simulink model "TB32_A25R_ClampMix"  (R2025a)
settings: Solver=FixedStepDiscrete  StartTime=0  StopTime=TB.t_end  FixedStep=TB.dt  RelTol=1e-3
InitFcn:
  | % 모델과 같은 폴더의 초기화 스크립트를 실행해 P(설계 파라미터)와 TB(시험 조건)를 만든다.
  | run(fullfile(fileparts(get_param(bdroot, 'FileName')), 'TB32_init.m'));
values from neighbouring files (symbols this model uses):
  TB = struct()    [TB32_init.m]    (also in run_TB32.m = evalin('base', 'TB'))
libraries: fl_lib x227, nesl_utility x83
(part 3 of 4)

== system TB32_A25R_ClampMix/StageC_Regulated/Primary_Bridge ==
  note: Stage C 1차 풀브리지(650 V GaN 2병렬): 1차가 보낼 때 250 kHz 50 % 상보 + 데드타임 t_dp, 2차가 보낼 때는 꺼 두고 다이오드 정류(경부하 두 브리지 구동 모드에서는 같은 위상)
  Q1_leg1_high : Subsystem  mask(PRISM-Hub switch cell){Ron=TB.CP.Ron, Goff=TB.CP.Goff, Vf=TB.CP.Vf, Rd=TB.CP.Rd, Goffd=TB.CP.Goffd, Coss=TB.CP.Coss}
      mask prompts: Ron "도통 저항 R_on [Ohm]"; Goff "차단 컨덕턴스 G_off [S]"; Vf "다이오드 순방향 전압 Vf [V]"; Rd "다이오드 도통 저항 R_d [Ohm]"; Goffd "다이오드 차단 컨덕턴스 [S]"; Coss "출력용량 C_oss [F]"
      mask help: 전력 반도체 스위치 셀 Q1_leg1_high. 게이트 태그 gC_Q1.
      settings: AttributesFormatString=gate: gC_Q1
      mask Display:
      | plot([0.50 0.50 ],[0.95 0.65 ],[0.50 0.74 ],[0.65 0.35 ],[0.50 0.50 ],[0.35 0.05 ]);
      | plot([0.50 0.20 0.20 ],[0.80 0.80 0.58 ],[0.20 0.20 0.50 ],[0.42 0.20 0.20 ]);
      | plot([0.20 0.10 0.30 0.20 ],[0.58 0.42 0.42 0.58 ],[0.10 0.30 ],[0.58 0.58 ]);
      | port_label('LConn',1,'D');
      | port_label('RConn',1,'S');
  Q2_leg1_low : Subsystem  mask(PRISM-Hub switch cell){Ron=TB.CP.Ron, Goff=TB.CP.Goff, Vf=TB.CP.Vf, Rd=TB.CP.Rd, Goffd=TB.CP.Goffd, Coss=TB.CP.Coss}
      mask prompts: Ron "도통 저항 R_on [Ohm]"; Goff "차단 컨덕턴스 G_off [S]"; Vf "다이오드 순방향 전압 Vf [V]"; Rd "다이오드 도통 저항 R_d [Ohm]"; Goffd "다이오드 차단 컨덕턴스 [S]"; Coss "출력용량 C_oss [F]"
      mask help: 전력 반도체 스위치 셀 Q2_leg1_low. 게이트 태그 gC_Q2.
      settings: AttributesFormatString=gate: gC_Q2
      mask Display:
      | plot([0.50 0.50 ],[0.95 0.65 ],[0.50 0.74 ],[0.65 0.35 ],[0.50 0.50 ],[0.35 0.05 ]);
      | plot([0.50 0.20 0.20 ],[0.80 0.80 0.58 ],[0.20 0.20 0.50 ],[0.42 0.20 0.20 ]);
      | plot([0.20 0.10 0.30 0.20 ],[0.58 0.42 0.42 0.58 ],[0.10 0.30 ],[0.58 0.58 ]);
      | port_label('LConn',1,'D');
      | port_label('RConn',1,'S');
  Q3_leg2_high : Subsystem  mask(PRISM-Hub switch cell){Ron=TB.CP.Ron, Goff=TB.CP.Goff, Vf=TB.CP.Vf, Rd=TB.CP.Rd, Goffd=TB.CP.Goffd, Coss=TB.CP.Coss}
      mask prompts: Ron "도통 저항 R_on [Ohm]"; Goff "차단 컨덕턴스 G_off [S]"; Vf "다이오드 순방향 전압 Vf [V]"; Rd "다이오드 도통 저항 R_d [Ohm]"; Goffd "다이오드 차단 컨덕턴스 [S]"; Coss "출력용량 C_oss [F]"
      mask help: 전력 반도체 스위치 셀 Q3_leg2_high. 게이트 태그 gC_Q3.
      settings: AttributesFormatString=gate: gC_Q3
      mask Display:
      | plot([0.50 0.50 ],[0.95 0.65 ],[0.50 0.74 ],[0.65 0.35 ],[0.50 0.50 ],[0.35 0.05 ]);
      | plot([0.50 0.20 0.20 ],[0.80 0.80 0.58 ],[0.20 0.20 0.50 ],[0.42 0.20 0.20 ]);
      | plot([0.20 0.10 0.30 0.20 ],[0.58 0.42 0.42 0.58 ],[0.10 0.30 ],[0.58 0.58 ]);
      | port_label('LConn',1,'D');
      | port_label('RConn',1,'S');
  Q4_leg2_low : Subsystem  mask(PRISM-Hub switch cell){Ron=TB.CP.Ron, Goff=TB.CP.Goff, Vf=TB.CP.Vf, Rd=TB.CP.Rd, Goffd=TB.CP.Goffd, Coss=TB.CP.Coss}
      mask prompts: Ron "도통 저항 R_on [Ohm]"; Goff "차단 컨덕턴스 G_off [S]"; Vf "다이오드 순방향 전압 Vf [V]"; Rd "다이오드 도통 저항 R_d [Ohm]"; Goffd "다이오드 차단 컨덕턴스 [S]"; Coss "출력용량 C_oss [F]"
      mask help: 전력 반도체 스위치 셀 Q4_leg2_low. 게이트 태그 gC_Q4.
      settings: AttributesFormatString=gate: gC_Q4
      mask Display:
      | plot([0.50 0.50 ],[0.95 0.65 ],[0.50 0.74 ],[0.65 0.35 ],[0.50 0.50 ],[0.35 0.05 ]);
      | plot([0.50 0.20 0.20 ],[0.80 0.80 0.58 ],[0.20 0.20 0.50 ],[0.42 0.20 0.20 ]);
      | plot([0.20 0.10 0.30 0.20 ],[0.58 0.42 0.42 0.58 ],[0.10 0.30 ],[0.58 0.58 ]);
      | port_label('LConn',1,'D');
      | port_label('RConn',1,'S');
  DC_P : PMIOPort  Side=Left
  DC_N : PMIOPort  Port=2  Side=Left
  AC1 : PMIOPort  Port=3  Side=Right
  AC2 : PMIOPort  Port=4  Side=Right
  connections:
  Q1_leg1_high/LConn1 -- DC_P/RConn1 -- Q3_leg2_high/LConn1
  Q2_leg1_low/LConn1 -- Q1_leg1_high/RConn1 -- AC1/RConn1
  Q4_leg2_low/LConn1 -- Q3_leg2_high/RConn1 -- AC2/RConn1
  DC_N/RConn1 -- Q2_leg1_low/RConn1 -- Q4_leg2_low/RConn1

== system TB32_A25R_ClampMix/StageC_Regulated/SB_H_high ==
  note: 스위치 셀: 이상 스위치(R_on, G_off) + 역병렬 바디 다이오드(Vf, R_d) + 출력용량 C_oss
      | 게이트: 전역 태그 "gS_BH" (> 0.5 이면 도통)
  C_oss : fl_lib/Electrical/Electrical Elements/Capacitor  c=Coss F  r=1e-6 Ohm  g=0 1/Ohm  i_specify=off  i_priority=None  i=0 A  i_nominal_specify=off  i_nominal_value=1  i_nominal_unit=A  v_specify=off  v_priority=None  v=0 V  v_nominal_specify=off  v_nominal_value=1  v_nominal_unit=V  vc_specify=off  vc_priority=High  vc=0 V  vc_nominal_specify=off  vc_nominal_value=1  vc_nominal_unit=V
  D_body : fl_lib/Electrical/Electrical Elements/Diode  Vf=Vf V  Ron=Rd Ohm  Goff=Goffd 1/Ohm  i_specify=off  i_priority=None  i=0 A  i_nominal_specify=off  i_nominal_value=1  i_nominal_unit=A  v_specify=off  v_priority=None  v=0 V  v_nominal_specify=off  v_nominal_value=1  v_nominal_unit=V
  Gate_PS : nesl_utility/Simulink-PS Converter  PhysicalDomain=network_engine_domain  SubClassName=ps_input  LeftPortType=input  RightPortType=output  PseudoPeriodic=off  Frequencies=[]  NoiseDistribution=none  NoiseParameters=[]  Unit=1  AffineConversion=off  FilteringAndDerivatives=zero  SimscapeFilterOrder=1  InputFilterTimeConstant=0.001  UdotUserProvided=0
  SW : fl_lib/Electrical/Electrical Elements/Switch  R_closed=Ron Ohm  G_open=Goff 1/Ohm  Threshold=0.5  i_specify=off  i_priority=None  i=0 A  i_nominal_specify=off  i_nominal_value=1  i_nominal_unit=A  v_specify=off  v_priority=None  v=0 V  v_nominal_specify=off  v_nominal_value=1  v_nominal_unit=V
  D : PMIOPort  Side=Left
  S : PMIOPort  Port=2  Side=Right
  wires:
  [gS_BH] -> Gate_PS/1
  connections:
  Gate_PS/RConn1 -- SW/RConn1
  SW/LConn1 -- D/RConn1 -- D_body/RConn1 -- C_oss/LConn1
  SW/RConn2 -- D_body/LConn1 -- S/RConn1 -- C_oss/RConn1

== system TB32_A25R_ClampMix/StageC_Regulated/SB_L_low ==
  note: 스위치 셀: 이상 스위치(R_on, G_off) + 역병렬 바디 다이오드(Vf, R_d) + 출력용량 C_oss
      | 게이트: 전역 태그 "gS_BL" (> 0.5 이면 도통)
  C_oss : fl_lib/Electrical/Electrical Elements/Capacitor  c=Coss F  r=1e-6 Ohm  g=0 1/Ohm  i_specify=off  i_priority=None  i=0 A  i_nominal_specify=off  i_nominal_value=1  i_nominal_unit=A  v_specify=off  v_priority=None  v=0 V  v_nominal_specify=off  v_nominal_value=1  v_nominal_unit=V  vc_specify=off  vc_priority=High  vc=0 V  vc_nominal_specify=off  vc_nominal_value=1  vc_nominal_unit=V
  D_body : fl_lib/Electrical/Electrical Elements/Diode  Vf=Vf V  Ron=Rd Ohm  Goff=Goffd 1/Ohm  i_specify=off  i_priority=None  i=0 A  i_nominal_specify=off  i_nominal_value=1  i_nominal_unit=A  v_specify=off  v_priority=None  v=0 V  v_nominal_specify=off  v_nominal_value=1  v_nominal_unit=V
  Gate_PS : nesl_utility/Simulink-PS Converter  PhysicalDomain=network_engine_domain  SubClassName=ps_input  LeftPortType=input  RightPortType=output  PseudoPeriodic=off  Frequencies=[]  NoiseDistribution=none  NoiseParameters=[]  Unit=1  AffineConversion=off  FilteringAndDerivatives=zero  SimscapeFilterOrder=1  InputFilterTimeConstant=0.001  UdotUserProvided=0
  SW : fl_lib/Electrical/Electrical Elements/Switch  R_closed=Ron Ohm  G_open=Goff 1/Ohm  Threshold=0.5  i_specify=off  i_priority=None  i=0 A  i_nominal_specify=off  i_nominal_value=1  i_nominal_unit=A  v_specify=off  v_priority=None  v=0 V  v_nominal_specify=off  v_nominal_value=1  v_nominal_unit=V
  D : PMIOPort  Side=Left
  S : PMIOPort  Port=2  Side=Right
  wires:
  [gS_BL] -> Gate_PS/1
  connections:
  Gate_PS/RConn1 -- SW/RConn1
  SW/LConn1 -- D/RConn1 -- D_body/RConn1 -- C_oss/LConn1
  SW/RConn2 -- D_body/LConn1 -- S/RConn1 -- C_oss/RConn1

== system TB32_A25R_ClampMix/StageC_Regulated/Secondary_Bridge ==
  note: Stage C 2차 풀브리지(150 V GaN 2병렬): 1차가 보낼 때는 꺼 두고 다이오드 정류(이상 동기정류 근사), 2차가 보낼 때 250 kHz + 데드타임 t_ds
  S1_leg1_high : Subsystem  mask(PRISM-Hub switch cell){Ron=TB.CS.Ron, Goff=TB.CS.Goff, Vf=TB.CS.Vf, Rd=TB.CS.Rd, Goffd=TB.CS.Goffd, Coss=TB.CS.Coss}
      mask prompts: Ron "도통 저항 R_on [Ohm]"; Goff "차단 컨덕턴스 G_off [S]"; Vf "다이오드 순방향 전압 Vf [V]"; Rd "다이오드 도통 저항 R_d [Ohm]"; Goffd "다이오드 차단 컨덕턴스 [S]"; Coss "출력용량 C_oss [F]"
      mask help: 전력 반도체 스위치 셀 S1_leg1_high. 게이트 태그 gC_S1.
      settings: AttributesFormatString=gate: gC_S1
      mask Display:
      | plot([0.50 0.50 ],[0.95 0.65 ],[0.50 0.74 ],[0.65 0.35 ],[0.50 0.50 ],[0.35 0.05 ]);
      | plot([0.50 0.20 0.20 ],[0.80 0.80 0.58 ],[0.20 0.20 0.50 ],[0.42 0.20 0.20 ]);
      | plot([0.20 0.10 0.30 0.20 ],[0.58 0.42 0.42 0.58 ],[0.10 0.30 ],[0.58 0.58 ]);
      | port_label('LConn',1,'D');
      | port_label('RConn',1,'S');
  S2_leg1_low : Subsystem  mask(PRISM-Hub switch cell){Ron=TB.CS.Ron, Goff=TB.CS.Goff, Vf=TB.CS.Vf, Rd=TB.CS.Rd, Goffd=TB.CS.Goffd, Coss=TB.CS.Coss}
      mask prompts: Ron "도통 저항 R_on [Ohm]"; Goff "차단 컨덕턴스 G_off [S]"; Vf "다이오드 순방향 전압 Vf [V]"; Rd "다이오드 도통 저항 R_d [Ohm]"; Goffd "다이오드 차단 컨덕턴스 [S]"; Coss "출력용량 C_oss [F]"
      mask help: 전력 반도체 스위치 셀 S2_leg1_low. 게이트 태그 gC_S2.
      settings: AttributesFormatString=gate: gC_S2
      mask Display:
      | plot([0.50 0.50 ],[0.95 0.65 ],[0.50 0.74 ],[0.65 0.35 ],[0.50 0.50 ],[0.35 0.05 ]);
      | plot([0.50 0.20 0.20 ],[0.80 0.80 0.58 ],[0.20 0.20 0.50 ],[0.42 0.20 0.20 ]);
      | plot([0.20 0.10 0.30 0.20 ],[0.58 0.42 0.42 0.58 ],[0.10 0.30 ],[0.58 0.58 ]);
      | port_label('LConn',1,'D');
      | port_label('RConn',1,'S');
  S3_leg2_high : Subsystem  mask(PRISM-Hub switch cell){Ron=TB.CS.Ron, Goff=TB.CS.Goff, Vf=TB.CS.Vf, Rd=TB.CS.Rd, Goffd=TB.CS.Goffd, Coss=TB.CS.Coss}
      mask prompts: Ron "도통 저항 R_on [Ohm]"; Goff "차단 컨덕턴스 G_off [S]"; Vf "다이오드 순방향 전압 Vf [V]"; Rd "다이오드 도통 저항 R_d [Ohm]"; Goffd "다이오드 차단 컨덕턴스 [S]"; Coss "출력용량 C_oss [F]"
      mask help: 전력 반도체 스위치 셀 S3_leg2_high. 게이트 태그 gC_S3.
      settings: AttributesFormatString=gate: gC_S3
      mask Display:
      | plot([0.50 0.50 ],[0.95 0.65 ],[0.50 0.74 ],[0.65 0.35 ],[0.50 0.50 ],[0.35 0.05 ]);
      | plot([0.50 0.20 0.20 ],[0.80 0.80 0.58 ],[0.20 0.20 0.50 ],[0.42 0.20 0.20 ]);
      | plot([0.20 0.10 0.30 0.20 ],[0.58 0.42 0.42 0.58 ],[0.10 0.30 ],[0.58 0.58 ]);
      | port_label('LConn',1,'D');
      | port_label('RConn',1,'S');
  S4_leg2_low : Subsystem  mask(PRISM-Hub switch cell){Ron=TB.CS.Ron, Goff=TB.CS.Goff, Vf=TB.CS.Vf, Rd=TB.CS.Rd, Goffd=TB.CS.Goffd, Coss=TB.CS.Coss}
      mask prompts: Ron "도통 저항 R_on [Ohm]"; Goff "차단 컨덕턴스 G_off [S]"; Vf "다이오드 순방향 전압 Vf [V]"; Rd "다이오드 도통 저항 R_d [Ohm]"; Goffd "다이오드 차단 컨덕턴스 [S]"; Coss "출력용량 C_oss [F]"
      mask help: 전력 반도체 스위치 셀 S4_leg2_low. 게이트 태그 gC_S4.
      settings: AttributesFormatString=gate: gC_S4
      mask Display:
      | plot([0.50 0.50 ],[0.95 0.65 ],[0.50 0.74 ],[0.65 0.35 ],[0.50 0.50 ],[0.35 0.05 ]);
      | plot([0.50 0.20 0.20 ],[0.80 0.80 0.58 ],[0.20 0.20 0.50 ],[0.42 0.20 0.20 ]);
      | plot([0.20 0.10 0.30 0.20 ],[0.58 0.42 0.42 0.58 ],[0.10 0.30 ],[0.58 0.58 ]);
      | port_label('LConn',1,'D');
      | port_label('RConn',1,'S');
  DC_P : PMIOPort  Side=Left
  DC_N : PMIOPort  Port=2  Side=Left
  AC1 : PMIOPort  Port=3  Side=Right
  AC2 : PMIOPort  Port=4  Side=Right
  connections:
  S1_leg1_high/LConn1 -- DC_P/RConn1 -- S3_leg2_high/LConn1
  S2_leg1_low/LConn1 -- S1_leg1_high/RConn1 -- AC1/RConn1
  S4_leg2_low/LConn1 -- S3_leg2_high/RConn1 -- AC2/RConn1
  DC_N/RConn1 -- S2_leg1_low/RConn1 -- S4_leg2_low/RConn1

== system TB32_A25R_ClampMix/StageA_Module1/StageA_Phase1/S1_VIN_A ==
  note: 스위치 셀: 이상 스위치(R_on, G_off) + 역병렬 바디 다이오드(Vf, R_d) + 출력용량 C_oss
      | 게이트: 전역 태그 "gA_P1_S1" (> 0.5 이면 도통)
  C_oss : fl_lib/Electrical/Electrical Elements/Capacitor  c=Coss F  r=1e-6 Ohm  g=0 1/Ohm  i_specify=off  i_priority=None  i=0 A  i_nominal_specify=off  i_nominal_value=1  i_nominal_unit=A  v_specify=off  v_priority=None  v=0 V  v_nominal_specify=off  v_nominal_value=1  v_nominal_unit=V  vc_specify=off  vc_priority=High  vc=0 V  vc_nominal_specify=off  vc_nominal_value=1  vc_nominal_unit=V
  D_body : fl_lib/Electrical/Electrical Elements/Diode  Vf=Vf V  Ron=Rd Ohm  Goff=Goffd 1/Ohm  i_specify=off  i_priority=None  i=0 A  i_nominal_specify=off  i_nominal_value=1  i_nominal_unit=A  v_specify=off  v_priority=None  v=0 V  v_nominal_specify=off  v_nominal_value=1  v_nominal_unit=V
  Gate_PS : nesl_utility/Simulink-PS Converter  PhysicalDomain=network_engine_domain  SubClassName=ps_input  LeftPortType=input  RightPortType=output  PseudoPeriodic=off  Frequencies=[]  NoiseDistribution=none  NoiseParameters=[]  Unit=1  AffineConversion=off  FilteringAndDerivatives=zero  SimscapeFilterOrder=1  InputFilterTimeConstant=0.001  UdotUserProvided=0
  SW : fl_lib/Electrical/Electrical Elements/Switch  R_closed=Ron Ohm  G_open=Goff 1/Ohm  Threshold=0.5  i_specify=off  i_priority=None  i=0 A  i_nominal_specify=off  i_nominal_value=1  i_nominal_unit=A  v_specify=off  v_priority=None  v=0 V  v_nominal_specify=off  v_nominal_value=1  v_nominal_unit=V
  D : PMIOPort  Side=Left
  S : PMIOPort  Port=2  Side=Right
  wires:
  [gA_P1_S1] -> Gate_PS/1
  connections:
  Gate_PS/RConn1 -- SW/RConn1
  SW/LConn1 -- D/RConn1 -- D_body/RConn1 -- C_oss/LConn1
  SW/RConn2 -- D_body/LConn1 -- S/RConn1 -- C_oss/RConn1

== system TB32_A25R_ClampMix/StageA_Module1/StageA_Phase1/S2_A_VOUT ==
  note: 스위치 셀: 이상 스위치(R_on, G_off) + 역병렬 바디 다이오드(Vf, R_d) + 출력용량 C_oss
      | 게이트: 전역 태그 "gA_P1_S2" (> 0.5 이면 도통)
  C_oss : fl_lib/Electrical/Electrical Elements/Capacitor  c=Coss F  r=1e-6 Ohm  g=0 1/Ohm  i_specify=off  i_priority=None  i=0 A  i_nominal_specify=off  i_nominal_value=1  i_nominal_unit=A  v_specify=off  v_priority=None  v=0 V  v_nominal_specify=off  v_nominal_value=1  v_nominal_unit=V  vc_specify=off  vc_priority=High  vc=0 V  vc_nominal_specify=off  vc_nominal_value=1  vc_nominal_unit=V
  D_body : fl_lib/Electrical/Electrical Elements/Diode  Vf=Vf V  Ron=Rd Ohm  Goff=Goffd 1/Ohm  i_specify=off  i_priority=None  i=0 A  i_nominal_specify=off  i_nominal_value=1  i_nominal_unit=A  v_specify=off  v_priority=None  v=0 V  v_nominal_specify=off  v_nominal_value=1  v_nominal_unit=V
  Gate_PS : nesl_utility/Simulink-PS Converter  PhysicalDomain=network_engine_domain  SubClassName=ps_input  LeftPortType=input  RightPortType=output  PseudoPeriodic=off  Frequencies=[]  NoiseDistribution=none  NoiseParameters=[]  Unit=1  AffineConversion=off  FilteringAndDerivatives=zero  SimscapeFilterOrder=1  InputFilterTimeConstant=0.001  UdotUserProvided=0
  SW : fl_lib/Electrical/Electrical Elements/Switch  R_closed=Ron Ohm  G_open=Goff 1/Ohm  Threshold=0.5  i_specify=off  i_priority=None  i=0 A  i_nominal_specify=off  i_nominal_value=1  i_nominal_unit=A  v_specify=off  v_priority=None  v=0 V  v_nominal_specify=off  v_nominal_value=1  v_nominal_unit=V
  D : PMIOPort  Side=Left
  S : PMIOPort  Port=2  Side=Right
  wires:
  [gA_P1_S2] -> Gate_PS/1
  connections:
  Gate_PS/RConn1 -- SW/RConn1
  SW/LConn1 -- D/RConn1 -- D_body/RConn1 -- C_oss/LConn1
  SW/RConn2 -- D_body/LConn1 -- S/RConn1 -- C_oss/RConn1

== system TB32_A25R_ClampMix/StageA_Module1/StageA_Phase1/S3_VOUT_B ==
  note: 스위치 셀: 이상 스위치(R_on, G_off) + 역병렬 바디 다이오드(Vf, R_d) + 출력용량 C_oss
      | 게이트: 전역 태그 "gA_P1_S3" (> 0.5 이면 도통)
  C_oss : fl_lib/Electrical/Electrical Elements/Capacitor  c=Coss F  r=1e-6 Ohm  g=0 1/Ohm  i_specify=off  i_priority=None  i=0 A  i_nominal_specify=off  i_nominal_value=1  i_nominal_unit=A  v_specify=off  v_priority=None  v=0 V  v_nominal_specify=off  v_nominal_value=1  v_nominal_unit=V  vc_specify=off  vc_priority=High  vc=0 V  vc_nominal_specify=off  vc_nominal_value=1  vc_nominal_unit=V
  D_body : fl_lib/Electrical/Electrical Elements/Diode  Vf=Vf V  Ron=Rd Ohm  Goff=Goffd 1/Ohm  i_specify=off  i_priority=None  i=0 A  i_nominal_specify=off  i_nominal_value=1  i_nominal_unit=A  v_specify=off  v_priority=None  v=0 V  v_nominal_specify=off  v_nominal_value=1  v_nominal_unit=V
  Gate_PS : nesl_utility/Simulink-PS Converter  PhysicalDomain=network_engine_domain  SubClassName=ps_input  LeftPortType=input  RightPortType=output  PseudoPeriodic=off  Frequencies=[]  NoiseDistribution=none  NoiseParameters=[]  Unit=1  AffineConversion=off  FilteringAndDerivatives=zero  SimscapeFilterOrder=1  InputFilterTimeConstant=0.001  UdotUserProvided=0
  SW : fl_lib/Electrical/Electrical Elements/Switch  R_closed=Ron Ohm  G_open=Goff 1/Ohm  Threshold=0.5  i_specify=off  i_priority=None  i=0 A  i_nominal_specify=off  i_nominal_value=1  i_nominal_unit=A  v_specify=off  v_priority=None  v=0 V  v_nominal_specify=off  v_nominal_value=1  v_nominal_unit=V
  D : PMIOPort  Side=Left
  S : PMIOPort  Port=2  Side=Right
  wires:
  [gA_P1_S3] -> Gate_PS/1
  connections:
  Gate_PS/RConn1 -- SW/RConn1
  SW/LConn1 -- D/RConn1 -- D_body/RConn1 -- C_oss/LConn1
  SW/RConn2 -- D_body/LConn1 -- S/RConn1 -- C_oss/RConn1

== system TB32_A25R_ClampMix/StageA_Module1/StageA_Phase1/S4_B_GND ==
  note: 스위치 셀: 이상 스위치(R_on, G_off) + 역병렬 바디 다이오드(Vf, R_d) + 출력용량 C_oss
      | 게이트: 전역 태그 "gA_P1_S4" (> 0.5 이면 도통)
  C_oss : fl_lib/Electrical/Electrical Elements/Capacitor  c=Coss F  r=1e-6 Ohm  g=0 1/Ohm  i_specify=off  i_priority=None  i=0 A  i_nominal_specify=off  i_nominal_value=1  i_nominal_unit=A  v_specify=off  v_priority=None  v=0 V  v_nominal_specify=off  v_nominal_value=1  v_nominal_unit=V  vc_specify=off  vc_priority=High  vc=0 V  vc_nominal_specify=off  vc_nominal_value=1  vc_nominal_unit=V
  D_body : fl_lib/Electrical/Electrical Elements/Diode  Vf=Vf V  Ron=Rd Ohm  Goff=Goffd 1/Ohm  i_specify=off  i_priority=None  i=0 A  i_nominal_specify=off  i_nominal_value=1  i_nominal_unit=A  v_specify=off  v_priority=None  v=0 V  v_nominal_specify=off  v_nominal_value=1  v_nominal_unit=V
  Gate_PS : nesl_utility/Simulink-PS Converter  PhysicalDomain=network_engine_domain  SubClassName=ps_input  LeftPortType=input  RightPortType=output  PseudoPeriodic=off  Frequencies=[]  NoiseDistribution=none  NoiseParameters=[]  Unit=1  AffineConversion=off  FilteringAndDerivatives=zero  SimscapeFilterOrder=1  InputFilterTimeConstant=0.001  UdotUserProvided=0
  SW : fl_lib/Electrical/Electrical Elements/Switch  R_closed=Ron Ohm  G_open=Goff 1/Ohm  Threshold=0.5  i_specify=off  i_priority=None  i=0 A  i_nominal_specify=off  i_nominal_value=1  i_nominal_unit=A  v_specify=off  v_priority=None  v=0 V  v_nominal_specify=off  v_nominal_value=1  v_nominal_unit=V
  D : PMIOPort  Side=Left
  S : PMIOPort  Port=2  Side=Right
  wires:
  [gA_P1_S4] -> Gate_PS/1
  connections:
  Gate_PS/RConn1 -- SW/RConn1
  SW/LConn1 -- D/RConn1 -- D_body/RConn1 -- C_oss/LConn1
  SW/RConn2 -- D_body/LConn1 -- S/RConn1 -- C_oss/RConn1

== system TB32_A25R_ClampMix/StageA_Module1/StageA_Phase2/S1_VIN_A ==
  note: 스위치 셀: 이상 스위치(R_on, G_off) + 역병렬 바디 다이오드(Vf, R_d) + 출력용량 C_oss
      | 게이트: 전역 태그 "gA_P2_S1" (> 0.5 이면 도통)
  C_oss : fl_lib/Electrical/Electrical Elements/Capacitor  c=Coss F  r=1e-6 Ohm  g=0 1/Ohm  i_specify=off  i_priority=None  i=0 A  i_nominal_specify=off  i_nominal_value=1  i_nominal_unit=A  v_specify=off  v_priority=None  v=0 V  v_nominal_specify=off  v_nominal_value=1  v_nominal_unit=V  vc_specify=off  vc_priority=High  vc=0 V  vc_nominal_specify=off  vc_nominal_value=1  vc_nominal_unit=V
  D_body : fl_lib/Electrical/Electrical Elements/Diode  Vf=Vf V  Ron=Rd Ohm  Goff=Goffd 1/Ohm  i_specify=off  i_priority=None  i=0 A  i_nominal_specify=off  i_nominal_value=1  i_nominal_unit=A  v_specify=off  v_priority=None  v=0 V  v_nominal_specify=off  v_nominal_value=1  v_nominal_unit=V
  Gate_PS : nesl_utility/Simulink-PS Converter  PhysicalDomain=network_engine_domain  SubClassName=ps_input  LeftPortType=input  RightPortType=output  PseudoPeriodic=off  Frequencies=[]  NoiseDistribution=none  NoiseParameters=[]  Unit=1  AffineConversion=off  FilteringAndDerivatives=zero  SimscapeFilterOrder=1  InputFilterTimeConstant=0.001  UdotUserProvided=0
  SW : fl_lib/Electrical/Electrical Elements/Switch  R_closed=Ron Ohm  G_open=Goff 1/Ohm  Threshold=0.5  i_specify=off  i_priority=None  i=0 A  i_nominal_specify=off  i_nominal_value=1  i_nominal_unit=A  v_specify=off  v_priority=None  v=0 V  v_nominal_specify=off  v_nominal_value=1  v_nominal_unit=V
  D : PMIOPort  Side=Left
  S : PMIOPort  Port=2  Side=Right
  wires:
  [gA_P2_S1] -> Gate_PS/1
  connections:
  Gate_PS/RConn1 -- SW/RConn1
  SW/LConn1 -- D/RConn1 -- D_body/RConn1 -- C_oss/LConn1
  SW/RConn2 -- D_body/LConn1 -- S/RConn1 -- C_oss/RConn1

== system TB32_A25R_ClampMix/StageA_Module1/StageA_Phase2/S2_A_VOUT ==
  note: 스위치 셀: 이상 스위치(R_on, G_off) + 역병렬 바디 다이오드(Vf, R_d) + 출력용량 C_oss
      | 게이트: 전역 태그 "gA_P2_S2" (> 0.5 이면 도통)
  C_oss : fl_lib/Electrical/Electrical Elements/Capacitor  c=Coss F  r=1e-6 Ohm  g=0 1/Ohm  i_specify=off  i_priority=None  i=0 A  i_nominal_specify=off  i_nominal_value=1  i_nominal_unit=A  v_specify=off  v_priority=None  v=0 V  v_nominal_specify=off  v_nominal_value=1  v_nominal_unit=V  vc_specify=off  vc_priority=High  vc=0 V  vc_nominal_specify=off  vc_nominal_value=1  vc_nominal_unit=V
  D_body : fl_lib/Electrical/Electrical Elements/Diode  Vf=Vf V  Ron=Rd Ohm  Goff=Goffd 1/Ohm  i_specify=off  i_priority=None  i=0 A  i_nominal_specify=off  i_nominal_value=1  i_nominal_unit=A  v_specify=off  v_priority=None  v=0 V  v_nominal_specify=off  v_nominal_value=1  v_nominal_unit=V
  Gate_PS : nesl_utility/Simulink-PS Converter  PhysicalDomain=network_engine_domain  SubClassName=ps_input  LeftPortType=input  RightPortType=output  PseudoPeriodic=off  Frequencies=[]  NoiseDistribution=none  NoiseParameters=[]  Unit=1  AffineConversion=off  FilteringAndDerivatives=zero  SimscapeFilterOrder=1  InputFilterTimeConstant=0.001  UdotUserProvided=0
  SW : fl_lib/Electrical/Electrical Elements/Switch  R_closed=Ron Ohm  G_open=Goff 1/Ohm  Threshold=0.5  i_specify=off  i_priority=None  i=0 A  i_nominal_specify=off  i_nominal_value=1  i_nominal_unit=A  v_specify=off  v_priority=None  v=0 V  v_nominal_specify=off  v_nominal_value=1  v_nominal_unit=V
  D : PMIOPort  Side=Left
  S : PMIOPort  Port=2  Side=Right
  wires:
  [gA_P2_S2] -> Gate_PS/1
  connections:
  Gate_PS/RConn1 -- SW/RConn1
  SW/LConn1 -- D/RConn1 -- D_body/RConn1 -- C_oss/LConn1
  SW/RConn2 -- D_body/LConn1 -- S/RConn1 -- C_oss/RConn1

== system TB32_A25R_ClampMix/StageA_Module1/StageA_Phase2/S3_VOUT_B ==
  note: 스위치 셀: 이상 스위치(R_on, G_off) + 역병렬 바디 다이오드(Vf, R_d) + 출력용량 C_oss
      | 게이트: 전역 태그 "gA_P2_S3" (> 0.5 이면 도통)
  C_oss : fl_lib/Electrical/Electrical Elements/Capacitor  c=Coss F  r=1e-6 Ohm  g=0 1/Ohm  i_specify=off  i_priority=None  i=0 A  i_nominal_specify=off  i_nominal_value=1  i_nominal_unit=A  v_specify=off  v_priority=None  v=0 V  v_nominal_specify=off  v_nominal_value=1  v_nominal_unit=V  vc_specify=off  vc_priority=High  vc=0 V  vc_nominal_specify=off  vc_nominal_value=1  vc_nominal_unit=V
  D_body : fl_lib/Electrical/Electrical Elements/Diode  Vf=Vf V  Ron=Rd Ohm  Goff=Goffd 1/Ohm  i_specify=off  i_priority=None  i=0 A  i_nominal_specify=off  i_nominal_value=1  i_nominal_unit=A  v_specify=off  v_priority=None  v=0 V  v_nominal_specify=off  v_nominal_value=1  v_nominal_unit=V
  Gate_PS : nesl_utility/Simulink-PS Converter  PhysicalDomain=network_engine_domain  SubClassName=ps_input  LeftPortType=input  RightPortType=output  PseudoPeriodic=off  Frequencies=[]  NoiseDistribution=none  NoiseParameters=[]  Unit=1  AffineConversion=off  FilteringAndDerivatives=zero  SimscapeFilterOrder=1  InputFilterTimeConstant=0.001  UdotUserProvided=0
  SW : fl_lib/Electrical/Electrical Elements/Switch  R_closed=Ron Ohm  G_open=Goff 1/Ohm  Threshold=0.5  i_specify=off  i_priority=None  i=0 A  i_nominal_specify=off  i_nominal_value=1  i_nominal_unit=A  v_specify=off  v_priority=None  v=0 V  v_nominal_specify=off  v_nominal_value=1  v_nominal_unit=V
  D : PMIOPort  Side=Left
  S : PMIOPort  Port=2  Side=Right
  wires:
  [gA_P2_S3] -> Gate_PS/1
  connections:
  Gate_PS/RConn1 -- SW/RConn1
  SW/LConn1 -- D/RConn1 -- D_body/RConn1 -- C_oss/LConn1
  SW/RConn2 -- D_body/LConn1 -- S/RConn1 -- C_oss/RConn1

== system TB32_A25R_ClampMix/StageA_Module1/StageA_Phase2/S4_B_GND ==
  note: 스위치 셀: 이상 스위치(R_on, G_off) + 역병렬 바디 다이오드(Vf, R_d) + 출력용량 C_oss
      | 게이트: 전역 태그 "gA_P2_S4" (> 0.5 이면 도통)
  C_oss : fl_lib/Electrical/Electrical Elements/Capacitor  c=Coss F  r=1e-6 Ohm  g=0 1/Ohm  i_specify=off  i_priority=None  i=0 A  i_nominal_specify=off  i_nominal_value=1  i_nominal_unit=A  v_specify=off  v_priority=None  v=0 V  v_nominal_specify=off  v_nominal_value=1  v_nominal_unit=V  vc_specify=off  vc_priority=High  vc=0 V  vc_nominal_specify=off  vc_nominal_value=1  vc_nominal_unit=V
  D_body : fl_lib/Electrical/Electrical Elements/Diode  Vf=Vf V  Ron=Rd Ohm  Goff=Goffd 1/Ohm  i_specify=off  i_priority=None  i=0 A  i_nominal_specify=off  i_nominal_value=1  i_nominal_unit=A  v_specify=off  v_priority=None  v=0 V  v_nominal_specify=off  v_nominal_value=1  v_nominal_unit=V
  Gate_PS : nesl_utility/Simulink-PS Converter  PhysicalDomain=network_engine_domain  SubClassName=ps_input  LeftPortType=input  RightPortType=output  PseudoPeriodic=off  Frequencies=[]  NoiseDistribution=none  NoiseParameters=[]  Unit=1  AffineConversion=off  FilteringAndDerivatives=zero  SimscapeFilterOrder=1  InputFilterTimeConstant=0.001  UdotUserProvided=0
  SW : fl_lib/Electrical/Electrical Elements/Switch  R_closed=Ron Ohm  G_open=Goff 1/Ohm  Threshold=0.5  i_specify=off  i_priority=None  i=0 A  i_nominal_specify=off  i_nominal_value=1  i_nominal_unit=A  v_specify=off  v_priority=None  v=0 V  v_nominal_specify=off  v_nominal_value=1  v_nominal_unit=V
  D : PMIOPort  Side=Left
  S : PMIOPort  Port=2  Side=Right
  wires:
  [gA_P2_S4] -> Gate_PS/1
  connections:
  Gate_PS/RConn1 -- SW/RConn1
  SW/LConn1 -- D/RConn1 -- D_body/RConn1 -- C_oss/LConn1
  SW/RConn2 -- D_body/LConn1 -- S/RConn1 -- C_oss/RConn1

== system TB32_A25R_ClampMix/StageA_Module2/StageA_Phase3/S1_VIN_A ==
  note: 스위치 셀: 이상 스위치(R_on, G_off) + 역병렬 바디 다이오드(Vf, R_d) + 출력용량 C_oss
      | 게이트: 전역 태그 "gA_P3_S1" (> 0.5 이면 도통)
  C_oss : fl_lib/Electrical/Electrical Elements/Capacitor  c=Coss F  r=1e-6 Ohm  g=0 1/Ohm  i_specify=off  i_priority=None  i=0 A  i_nominal_specify=off  i_nominal_value=1  i_nominal_unit=A  v_specify=off  v_priority=None  v=0 V  v_nominal_specify=off  v_nominal_value=1  v_nominal_unit=V  vc_specify=off  vc_priority=High  vc=0 V  vc_nominal_specify=off  vc_nominal_value=1  vc_nominal_unit=V
  D_body : fl_lib/Electrical/Electrical Elements/Diode  Vf=Vf V  Ron=Rd Ohm  Goff=Goffd 1/Ohm  i_specify=off  i_priority=None  i=0 A  i_nominal_specify=off  i_nominal_value=1  i_nominal_unit=A  v_specify=off  v_priority=None  v=0 V  v_nominal_specify=off  v_nominal_value=1  v_nominal_unit=V
  Gate_PS : nesl_utility/Simulink-PS Converter  PhysicalDomain=network_engine_domain  SubClassName=ps_input  LeftPortType=input  RightPortType=output  PseudoPeriodic=off  Frequencies=[]  NoiseDistribution=none  NoiseParameters=[]  Unit=1  AffineConversion=off  FilteringAndDerivatives=zero  SimscapeFilterOrder=1  InputFilterTimeConstant=0.001  UdotUserProvided=0
  SW : fl_lib/Electrical/Electrical Elements/Switch  R_closed=Ron Ohm  G_open=Goff 1/Ohm  Threshold=0.5  i_specify=off  i_priority=None  i=0 A  i_nominal_specify=off  i_nominal_value=1  i_nominal_unit=A  v_specify=off  v_priority=None  v=0 V  v_nominal_specify=off  v_nominal_value=1  v_nominal_unit=V
  D : PMIOPort  Side=Left
  S : PMIOPort  Port=2  Side=Right
  wires:
  [gA_P3_S1] -> Gate_PS/1
  connections:
  Gate_PS/RConn1 -- SW/RConn1
  SW/LConn1 -- D/RConn1 -- D_body/RConn1 -- C_oss/LConn1
  SW/RConn2 -- D_body/LConn1 -- S/RConn1 -- C_oss/RConn1

== system TB32_A25R_ClampMix/StageA_Module2/StageA_Phase3/S2_A_VOUT ==
  note: 스위치 셀: 이상 스위치(R_on, G_off) + 역병렬 바디 다이오드(Vf, R_d) + 출력용량 C_oss
      | 게이트: 전역 태그 "gA_P3_S2" (> 0.5 이면 도통)
  C_oss : fl_lib/Electrical/Electrical Elements/Capacitor  c=Coss F  r=1e-6 Ohm  g=0 1/Ohm  i_specify=off  i_priority=None  i=0 A  i_nominal_specify=off  i_nominal_value=1  i_nominal_unit=A  v_specify=off  v_priority=None  v=0 V  v_nominal_specify=off  v_nominal_value=1  v_nominal_unit=V  vc_specify=off  vc_priority=High  vc=0 V  vc_nominal_specify=off  vc_nominal_value=1  vc_nominal_unit=V
  D_body : fl_lib/Electrical/Electrical Elements/Diode  Vf=Vf V  Ron=Rd Ohm  Goff=Goffd 1/Ohm  i_specify=off  i_priority=None  i=0 A  i_nominal_specify=off  i_nominal_value=1  i_nominal_unit=A  v_specify=off  v_priority=None  v=0 V  v_nominal_specify=off  v_nominal_value=1  v_nominal_unit=V
  Gate_PS : nesl_utility/Simulink-PS Converter  PhysicalDomain=network_engine_domain  SubClassName=ps_input  LeftPortType=input  RightPortType=output  PseudoPeriodic=off  Frequencies=[]  NoiseDistribution=none  NoiseParameters=[]  Unit=1  AffineConversion=off  FilteringAndDerivatives=zero  SimscapeFilterOrder=1  InputFilterTimeConstant=0.001  UdotUserProvided=0
  SW : fl_lib/Electrical/Electrical Elements/Switch  R_closed=Ron Ohm  G_open=Goff 1/Ohm  Threshold=0.5  i_specify=off  i_priority=None  i=0 A  i_nominal_specify=off  i_nominal_value=1  i_nominal_unit=A  v_specify=off  v_priority=None  v=0 V  v_nominal_specify=off  v_nominal_value=1  v_nominal_unit=V
  D : PMIOPort  Side=Left
  S : PMIOPort  Port=2  Side=Right
  wires:
  [gA_P3_S2] -> Gate_PS/1
  connections:
  Gate_PS/RConn1 -- SW/RConn1
  SW/LConn1 -- D/RConn1 -- D_body/RConn1 -- C_oss/LConn1
  SW/RConn2 -- D_body/LConn1 -- S/RConn1 -- C_oss/RConn1

== system TB32_A25R_ClampMix/StageA_Module2/StageA_Phase3/S3_VOUT_B ==
  note: 스위치 셀: 이상 스위치(R_on, G_off) + 역병렬 바디 다이오드(Vf, R_d) + 출력용량 C_oss
      | 게이트: 전역 태그 "gA_P3_S3" (> 0.5 이면 도통)
  C_oss : fl_lib/Electrical/Electrical Elements/Capacitor  c=Coss F  r=1e-6 Ohm  g=0 1/Ohm  i_specify=off  i_priority=None  i=0 A  i_nominal_specify=off  i_nominal_value=1  i_nominal_unit=A  v_specify=off  v_priority=None  v=0 V  v_nominal_specify=off  v_nominal_value=1  v_nominal_unit=V  vc_specify=off  vc_priority=High  vc=0 V  vc_nominal_specify=off  vc_nominal_value=1  vc_nominal_unit=V
  D_body : fl_lib/Electrical/Electrical Elements/Diode  Vf=Vf V  Ron=Rd Ohm  Goff=Goffd 1/Ohm  i_specify=off  i_priority=None  i=0 A  i_nominal_specify=off  i_nominal_value=1  i_nominal_unit=A  v_specify=off  v_priority=None  v=0 V  v_nominal_specify=off  v_nominal_value=1  v_nominal_unit=V
  Gate_PS : nesl_utility/Simulink-PS Converter  PhysicalDomain=network_engine_domain  SubClassName=ps_input  LeftPortType=input  RightPortType=output  PseudoPeriodic=off  Frequencies=[]  NoiseDistribution=none  NoiseParameters=[]  Unit=1  AffineConversion=off  FilteringAndDerivatives=zero  SimscapeFilterOrder=1  InputFilterTimeConstant=0.001  UdotUserProvided=0
  SW : fl_lib/Electrical/Electrical Elements/Switch  R_closed=Ron Ohm  G_open=Goff 1/Ohm  Threshold=0.5  i_specify=off  i_priority=None  i=0 A  i_nominal_specify=off  i_nominal_value=1  i_nominal_unit=A  v_specify=off  v_priority=None  v=0 V  v_nominal_specify=off  v_nominal_value=1  v_nominal_unit=V
  D : PMIOPort  Side=Left
  S : PMIOPort  Port=2  Side=Right
  wires:
  [gA_P3_S3] -> Gate_PS/1
  connections:
  Gate_PS/RConn1 -- SW/RConn1
  SW/LConn1 -- D/RConn1 -- D_body/RConn1 -- C_oss/LConn1
  SW/RConn2 -- D_body/LConn1 -- S/RConn1 -- C_oss/RConn1

== system TB32_A25R_ClampMix/StageA_Module2/StageA_Phase3/S4_B_GND ==
  note: 스위치 셀: 이상 스위치(R_on, G_off) + 역병렬 바디 다이오드(Vf, R_d) + 출력용량 C_oss
      | 게이트: 전역 태그 "gA_P3_S4" (> 0.5 이면 도통)
  C_oss : fl_lib/Electrical/Electrical Elements/Capacitor  c=Coss F  r=1e-6 Ohm  g=0 1/Ohm  i_specify=off  i_priority=None  i=0 A  i_nominal_specify=off  i_nominal_value=1  i_nominal_unit=A  v_specify=off  v_priority=None  v=0 V  v_nominal_specify=off  v_nominal_value=1  v_nominal_unit=V  vc_specify=off  vc_priority=High  vc=0 V  vc_nominal_specify=off  vc_nominal_value=1  vc_nominal_unit=V
  D_body : fl_lib/Electrical/Electrical Elements/Diode  Vf=Vf V  Ron=Rd Ohm  Goff=Goffd 1/Ohm  i_specify=off  i_priority=None  i=0 A  i_nominal_specify=off  i_nominal_value=1  i_nominal_unit=A  v_specify=off  v_priority=None  v=0 V  v_nominal_specify=off  v_nominal_value=1  v_nominal_unit=V
  Gate_PS : nesl_utility/Simulink-PS Converter  PhysicalDomain=network_engine_domain  SubClassName=ps_input  LeftPortType=input  RightPortType=output  PseudoPeriodic=off  Frequencies=[]  NoiseDistribution=none  NoiseParameters=[]  Unit=1  AffineConversion=off  FilteringAndDerivatives=zero  SimscapeFilterOrder=1  InputFilterTimeConstant=0.001  UdotUserProvided=0
  SW : fl_lib/Electrical/Electrical Elements/Switch  R_closed=Ron Ohm  G_open=Goff 1/Ohm  Threshold=0.5  i_specify=off  i_priority=None  i=0 A  i_nominal_specify=off  i_nominal_value=1  i_nominal_unit=A  v_specify=off  v_priority=None  v=0 V  v_nominal_specify=off  v_nominal_value=1  v_nominal_unit=V
  D : PMIOPort  Side=Left
  S : PMIOPort  Port=2  Side=Right
  wires:
  [gA_P3_S4] -> Gate_PS/1
  connections:
  Gate_PS/RConn1 -- SW/RConn1
  SW/LConn1 -- D/RConn1 -- D_body/RConn1 -- C_oss/LConn1
  SW/RConn2 -- D_body/LConn1 -- S/RConn1 -- C_oss/RConn1

== system TB32_A25R_ClampMix/StageA_Module2/StageA_Phase4/S1_VIN_A ==
  note: 스위치 셀: 이상 스위치(R_on, G_off) + 역병렬 바디 다이오드(Vf, R_d) + 출력용량 C_oss
      | 게이트: 전역 태그 "gA_P4_S1" (> 0.5 이면 도통)
  C_oss : fl_lib/Electrical/Electrical Elements/Capacitor  c=Coss F  r=1e-6 Ohm  g=0 1/Ohm  i_specify=off  i_priority=None  i=0 A  i_nominal_specify=off  i_nominal_value=1  i_nominal_unit=A  v_specify=off  v_priority=None  v=0 V  v_nominal_specify=off  v_nominal_value=1  v_nominal_unit=V  vc_specify=off  vc_priority=High  vc=0 V  vc_nominal_specify=off  vc_nominal_value=1  vc_nominal_unit=V
  D_body : fl_lib/Electrical/Electrical Elements/Diode  Vf=Vf V  Ron=Rd Ohm  Goff=Goffd 1/Ohm  i_specify=off  i_priority=None  i=0 A  i_nominal_specify=off  i_nominal_value=1  i_nominal_unit=A  v_specify=off  v_priority=None  v=0 V  v_nominal_specify=off  v_nominal_value=1  v_nominal_unit=V
  Gate_PS : nesl_utility/Simulink-PS Converter  PhysicalDomain=network_engine_domain  SubClassName=ps_input  LeftPortType=input  RightPortType=output  PseudoPeriodic=off  Frequencies=[]  NoiseDistribution=none  NoiseParameters=[]  Unit=1  AffineConversion=off  FilteringAndDerivatives=zero  SimscapeFilterOrder=1  InputFilterTimeConstant=0.001  UdotUserProvided=0
  SW : fl_lib/Electrical/Electrical Elements/Switch  R_closed=Ron Ohm  G_open=Goff 1/Ohm  Threshold=0.5  i_specify=off  i_priority=None  i=0 A  i_nominal_specify=off  i_nominal_value=1  i_nominal_unit=A  v_specify=off  v_priority=None  v=0 V  v_nominal_specify=off  v_nominal_value=1  v_nominal_unit=V
  D : PMIOPort  Side=Left
  S : PMIOPort  Port=2  Side=Right
  wires:
  [gA_P4_S1] -> Gate_PS/1
  connections:
  Gate_PS/RConn1 -- SW/RConn1
  SW/LConn1 -- D/RConn1 -- D_body/RConn1 -- C_oss/LConn1
  SW/RConn2 -- D_body/LConn1 -- S/RConn1 -- C_oss/RConn1

== system TB32_A25R_ClampMix/StageA_Module2/StageA_Phase4/S2_A_VOUT ==
  note: 스위치 셀: 이상 스위치(R_on, G_off) + 역병렬 바디 다이오드(Vf, R_d) + 출력용량 C_oss
      | 게이트: 전역 태그 "gA_P4_S2" (> 0.5 이면 도통)
  C_oss : fl_lib/Electrical/Electrical Elements/Capacitor  c=Coss F  r=1e-6 Ohm  g=0 1/Ohm  i_specify=off  i_priority=None  i=0 A  i_nominal_specify=off  i_nominal_value=1  i_nominal_unit=A  v_specify=off  v_priority=None  v=0 V  v_nominal_specify=off  v_nominal_value=1  v_nominal_unit=V  vc_specify=off  vc_priority=High  vc=0 V  vc_nominal_specify=off  vc_nominal_value=1  vc_nominal_unit=V
  D_body : fl_lib/Electrical/Electrical Elements/Diode  Vf=Vf V  Ron=Rd Ohm  Goff=Goffd 1/Ohm  i_specify=off  i_priority=None  i=0 A  i_nominal_specify=off  i_nominal_value=1  i_nominal_unit=A  v_specify=off  v_priority=None  v=0 V  v_nominal_specify=off  v_nominal_value=1  v_nominal_unit=V
  Gate_PS : nesl_utility/Simulink-PS Converter  PhysicalDomain=network_engine_domain  SubClassName=ps_input  LeftPortType=input  RightPortType=output  PseudoPeriodic=off  Frequencies=[]  NoiseDistribution=none  NoiseParameters=[]  Unit=1  AffineConversion=off  FilteringAndDerivatives=zero  SimscapeFilterOrder=1  InputFilterTimeConstant=0.001  UdotUserProvided=0
  SW : fl_lib/Electrical/Electrical Elements/Switch  R_closed=Ron Ohm  G_open=Goff 1/Ohm  Threshold=0.5  i_specify=off  i_priority=None  i=0 A  i_nominal_specify=off  i_nominal_value=1  i_nominal_unit=A  v_specify=off  v_priority=None  v=0 V  v_nominal_specify=off  v_nominal_value=1  v_nominal_unit=V
  D : PMIOPort  Side=Left
  S : PMIOPort  Port=2  Side=Right
  wires:
  [gA_P4_S2] -> Gate_PS/1
  connections:
  Gate_PS/RConn1 -- SW/RConn1
  SW/LConn1 -- D/RConn1 -- D_body/RConn1 -- C_oss/LConn1
  SW/RConn2 -- D_body/LConn1 -- S/RConn1 -- C_oss/RConn1

== system TB32_A25R_ClampMix/StageA_Module2/StageA_Phase4/S3_VOUT_B ==
  note: 스위치 셀: 이상 스위치(R_on, G_off) + 역병렬 바디 다이오드(Vf, R_d) + 출력용량 C_oss
      | 게이트: 전역 태그 "gA_P4_S3" (> 0.5 이면 도통)
  C_oss : fl_lib/Electrical/Electrical Elements/Capacitor  c=Coss F  r=1e-6 Ohm  g=0 1/Ohm  i_specify=off  i_priority=None  i=0 A  i_nominal_specify=off  i_nominal_value=1  i_nominal_unit=A  v_specify=off  v_priority=None  v=0 V  v_nominal_specify=off  v_nominal_value=1  v_nominal_unit=V  vc_specify=off  vc_priority=High  vc=0 V  vc_nominal_specify=off  vc_nominal_value=1  vc_nominal_unit=V
  D_body : fl_lib/Electrical/Electrical Elements/Diode  Vf=Vf V  Ron=Rd Ohm  Goff=Goffd 1/Ohm  i_specify=off  i_priority=None  i=0 A  i_nominal_specify=off  i_nominal_value=1  i_nominal_unit=A  v_specify=off  v_priority=None  v=0 V  v_nominal_specify=off  v_nominal_value=1  v_nominal_unit=V
  Gate_PS : nesl_utility/Simulink-PS Converter  PhysicalDomain=network_engine_domain  SubClassName=ps_input  LeftPortType=input  RightPortType=output  PseudoPeriodic=off  Frequencies=[]  NoiseDistribution=none  NoiseParameters=[]  Unit=1  AffineConversion=off  FilteringAndDerivatives=zero  SimscapeFilterOrder=1  InputFilterTimeConstant=0.001  UdotUserProvided=0
  SW : fl_lib/Electrical/Electrical Elements/Switch  R_closed=Ron Ohm  G_open=Goff 1/Ohm  Threshold=0.5  i_specify=off  i_priority=None  i=0 A  i_nominal_specify=off  i_nominal_value=1  i_nominal_unit=A  v_specify=off  v_priority=None  v=0 V  v_nominal_specify=off  v_nominal_value=1  v_nominal_unit=V
  D : PMIOPort  Side=Left
  S : PMIOPort  Port=2  Side=Right
  wires:
  [gA_P4_S3] -> Gate_PS/1
  connections:
  Gate_PS/RConn1 -- SW/RConn1
  SW/LConn1 -- D/RConn1 -- D_body/RConn1 -- C_oss/LConn1
  SW/RConn2 -- D_body/LConn1 -- S/RConn1 -- C_oss/RConn1

== system TB32_A25R_ClampMix/StageA_Module2/StageA_Phase4/S4_B_GND ==
  note: 스위치 셀: 이상 스위치(R_on, G_off) + 역병렬 바디 다이오드(Vf, R_d) + 출력용량 C_oss
      | 게이트: 전역 태그 "gA_P4_S4" (> 0.5 이면 도통)
  C_oss : fl_lib/Electrical/Electrical Elements/Capacitor  c=Coss F  r=1e-6 Ohm  g=0 1/Ohm  i_specify=off  i_priority=None  i=0 A  i_nominal_specify=off  i_nominal_value=1  i_nominal_unit=A  v_specify=off  v_priority=None  v=0 V  v_nominal_specify=off  v_nominal_value=1  v_nominal_unit=V  vc_specify=off  vc_priority=High  vc=0 V  vc_nominal_specify=off  vc_nominal_value=1  vc_nominal_unit=V
  D_body : fl_lib/Electrical/Electrical Elements/Diode  Vf=Vf V  Ron=Rd Ohm  Goff=Goffd 1/Ohm  i_specify=off  i_priority=None  i=0 A  i_nominal_specify=off  i_nominal_value=1  i_nominal_unit=A  v_specify=off  v_priority=None  v=0 V  v_nominal_specify=off  v_nominal_value=1  v_nominal_unit=V
  Gate_PS : nesl_utility/Simulink-PS Converter  PhysicalDomain=network_engine_domain  SubClassName=ps_input  LeftPortType=input  RightPortType=output  PseudoPeriodic=off  Frequencies=[]  NoiseDistribution=none  NoiseParameters=[]  Unit=1  AffineConversion=off  FilteringAndDerivatives=zero  SimscapeFilterOrder=1  InputFilterTimeConstant=0.001  UdotUserProvided=0
  SW : fl_lib/Electrical/Electrical Elements/Switch  R_closed=Ron Ohm  G_open=Goff 1/Ohm  Threshold=0.5  i_specify=off  i_priority=None  i=0 A  i_nominal_specify=off  i_nominal_value=1  i_nominal_unit=A  v_specify=off  v_priority=None  v=0 V  v_nominal_specify=off  v_nominal_value=1  v_nominal_unit=V
  D : PMIOPort  Side=Left
  S : PMIOPort  Port=2  Side=Right
  wires:
  [gA_P4_S4] -> Gate_PS/1
  connections:
  Gate_PS/RConn1 -- SW/RConn1
  SW/LConn1 -- D/RConn1 -- D_body/RConn1 -- C_oss/LConn1
  SW/RConn2 -- D_body/LConn1 -- S/RConn1 -- C_oss/RConn1

== system TB32_A25R_ClampMix/StageA_Module3/StageA_Phase5/S1_VIN_A ==
  note: 스위치 셀: 이상 스위치(R_on, G_off) + 역병렬 바디 다이오드(Vf, R_d) + 출력용량 C_oss
      | 게이트: 전역 태그 "gA_P5_S1" (> 0.5 이면 도통)
  C_oss : fl_lib/Electrical/Electrical Elements/Capacitor  c=Coss F  r=1e-6 Ohm  g=0 1/Ohm  i_specify=off  i_priority=None  i=0 A  i_nominal_specify=off  i_nominal_value=1  i_nominal_unit=A  v_specify=off  v_priority=None  v=0 V  v_nominal_specify=off  v_nominal_value=1  v_nominal_unit=V  vc_specify=off  vc_priority=High  vc=0 V  vc_nominal_specify=off  vc_nominal_value=1  vc_nominal_unit=V
  D_body : fl_lib/Electrical/Electrical Elements/Diode  Vf=Vf V  Ron=Rd Ohm  Goff=Goffd 1/Ohm  i_specify=off  i_priority=None  i=0 A  i_nominal_specify=off  i_nominal_value=1  i_nominal_unit=A  v_specify=off  v_priority=None  v=0 V  v_nominal_specify=off  v_nominal_value=1  v_nominal_unit=V
  Gate_PS : nesl_utility/Simulink-PS Converter  PhysicalDomain=network_engine_domain  SubClassName=ps_input  LeftPortType=input  RightPortType=output  PseudoPeriodic=off  Frequencies=[]  NoiseDistribution=none  NoiseParameters=[]  Unit=1  AffineConversion=off  FilteringAndDerivatives=zero  SimscapeFilterOrder=1  InputFilterTimeConstant=0.001  UdotUserProvided=0
  SW : fl_lib/Electrical/Electrical Elements/Switch  R_closed=Ron Ohm  G_open=Goff 1/Ohm  Threshold=0.5  i_specify=off  i_priority=None  i=0 A  i_nominal_specify=off  i_nominal_value=1  i_nominal_unit=A  v_specify=off  v_priority=None  v=0 V  v_nominal_specify=off  v_nominal_value=1  v_nominal_unit=V
  D : PMIOPort  Side=Left
  S : PMIOPort  Port=2  Side=Right
  wires:
  [gA_P5_S1] -> Gate_PS/1
  connections:
  Gate_PS/RConn1 -- SW/RConn1
  SW/LConn1 -- D/RConn1 -- D_body/RConn1 -- C_oss/LConn1
  SW/RConn2 -- D_body/LConn1 -- S/RConn1 -- C_oss/RConn1

== system TB32_A25R_ClampMix/StageA_Module3/StageA_Phase5/S2_A_VOUT ==
  note: 스위치 셀: 이상 스위치(R_on, G_off) + 역병렬 바디 다이오드(Vf, R_d) + 출력용량 C_oss
      | 게이트: 전역 태그 "gA_P5_S2" (> 0.5 이면 도통)
  C_oss : fl_lib/Electrical/Electrical Elements/Capacitor  c=Coss F  r=1e-6 Ohm  g=0 1/Ohm  i_specify=off  i_priority=None  i=0 A  i_nominal_specify=off  i_nominal_value=1  i_nominal_unit=A  v_specify=off  v_priority=None  v=0 V  v_nominal_specify=off  v_nominal_value=1  v_nominal_unit=V  vc_specify=off  vc_priority=High  vc=0 V  vc_nominal_specify=off  vc_nominal_value=1  vc_nominal_unit=V
  D_body : fl_lib/Electrical/Electrical Elements/Diode  Vf=Vf V  Ron=Rd Ohm  Goff=Goffd 1/Ohm  i_specify=off  i_priority=None  i=0 A  i_nominal_specify=off  i_nominal_value=1  i_nominal_unit=A  v_specify=off  v_priority=None  v=0 V  v_nominal_specify=off  v_nominal_value=1  v_nominal_unit=V
  Gate_PS : nesl_utility/Simulink-PS Converter  PhysicalDomain=network_engine_domain  SubClassName=ps_input  LeftPortType=input  RightPortType=output  PseudoPeriodic=off  Frequencies=[]  NoiseDistribution=none  NoiseParameters=[]  Unit=1  AffineConversion=off  FilteringAndDerivatives=zero  SimscapeFilterOrder=1  InputFilterTimeConstant=0.001  UdotUserProvided=0
  SW : fl_lib/Electrical/Electrical Elements/Switch  R_closed=Ron Ohm  G_open=Goff 1/Ohm  Threshold=0.5  i_specify=off  i_priority=None  i=0 A  i_nominal_specify=off  i_nominal_value=1  i_nominal_unit=A  v_specify=off  v_priority=None  v=0 V  v_nominal_specify=off  v_nominal_value=1  v_nominal_unit=V
  D : PMIOPort  Side=Left
  S : PMIOPort  Port=2  Side=Right
  wires:
  [gA_P5_S2] -> Gate_PS/1
  connections:
  Gate_PS/RConn1 -- SW/RConn1
  SW/LConn1 -- D/RConn1 -- D_body/RConn1 -- C_oss/LConn1
  SW/RConn2 -- D_body/LConn1 -- S/RConn1 -- C_oss/RConn1

== system TB32_A25R_ClampMix/StageA_Module3/StageA_Phase5/S3_VOUT_B ==
  note: 스위치 셀: 이상 스위치(R_on, G_off) + 역병렬 바디 다이오드(Vf, R_d) + 출력용량 C_oss
      | 게이트: 전역 태그 "gA_P5_S3" (> 0.5 이면 도통)
  C_oss : fl_lib/Electrical/Electrical Elements/Capacitor  c=Coss F  r=1e-6 Ohm  g=0 1/Ohm  i_specify=off  i_priority=None  i=0 A  i_nominal_specify=off  i_nominal_value=1  i_nominal_unit=A  v_specify=off  v_priority=None  v=0 V  v_nominal_specify=off  v_nominal_value=1  v_nominal_unit=V  vc_specify=off  vc_priority=High  vc=0 V  vc_nominal_specify=off  vc_nominal_value=1  vc_nominal_unit=V
  D_body : fl_lib/Electrical/Electrical Elements/Diode  Vf=Vf V  Ron=Rd Ohm  Goff=Goffd 1/Ohm  i_specify=off  i_priority=None  i=0 A  i_nominal_specify=off  i_nominal_value=1  i_nominal_unit=A  v_specify=off  v_priority=None  v=0 V  v_nominal_specify=off  v_nominal_value=1  v_nominal_unit=V
  Gate_PS : nesl_utility/Simulink-PS Converter  PhysicalDomain=network_engine_domain  SubClassName=ps_input  LeftPortType=input  RightPortType=output  PseudoPeriodic=off  Frequencies=[]  NoiseDistribution=none  NoiseParameters=[]  Unit=1  AffineConversion=off  FilteringAndDerivatives=zero  SimscapeFilterOrder=1  InputFilterTimeConstant=0.001  UdotUserProvided=0
  SW : fl_lib/Electrical/Electrical Elements/Switch  R_closed=Ron Ohm  G_open=Goff 1/Ohm  Threshold=0.5  i_specify=off  i_priority=None  i=0 A  i_nominal_specify=off  i_nominal_value=1  i_nominal_unit=A  v_specify=off  v_priority=None  v=0 V  v_nominal_specify=off  v_nominal_value=1  v_nominal_unit=V
  D : PMIOPort  Side=Left
  S : PMIOPort  Port=2  Side=Right
  wires:
  [gA_P5_S3] -> Gate_PS/1
  connections:
  Gate_PS/RConn1 -- SW/RConn1
  SW/LConn1 -- D/RConn1 -- D_body/RConn1 -- C_oss/LConn1
  SW/RConn2 -- D_body/LConn1 -- S/RConn1 -- C_oss/RConn1

== system TB32_A25R_ClampMix/StageA_Module3/StageA_Phase5/S4_B_GND ==
  note: 스위치 셀: 이상 스위치(R_on, G_off) + 역병렬 바디 다이오드(Vf, R_d) + 출력용량 C_oss
      | 게이트: 전역 태그 "gA_P5_S4" (> 0.5 이면 도통)
  C_oss : fl_lib/Electrical/Electrical Elements/Capacitor  c=Coss F  r=1e-6 Ohm  g=0 1/Ohm  i_specify=off  i_priority=None  i=0 A  i_nominal_specify=off  i_nominal_value=1  i_nominal_unit=A  v_specify=off  v_priority=None  v=0 V  v_nominal_specify=off  v_nominal_value=1  v_nominal_unit=V  vc_specify=off  vc_priority=High  vc=0 V  vc_nominal_specify=off  vc_nominal_value=1  vc_nominal_unit=V
  D_body : fl_lib/Electrical/Electrical Elements/Diode  Vf=Vf V  Ron=Rd Ohm  Goff=Goffd 1/Ohm  i_specify=off  i_priority=None  i=0 A  i_nominal_specify=off  i_nominal_value=1  i_nominal_unit=A  v_specify=off  v_priority=None  v=0 V  v_nominal_specify=off  v_nominal_value=1  v_nominal_unit=V
  Gate_PS : nesl_utility/Simulink-PS Converter  PhysicalDomain=network_engine_domain  SubClassName=ps_input  LeftPortType=input  RightPortType=output  PseudoPeriodic=off  Frequencies=[]  NoiseDistribution=none  NoiseParameters=[]  Unit=1  AffineConversion=off  FilteringAndDerivatives=zero  SimscapeFilterOrder=1  InputFilterTimeConstant=0.001  UdotUserProvided=0
  SW : fl_lib/Electrical/Electrical Elements/Switch  R_closed=Ron Ohm  G_open=Goff 1/Ohm  Threshold=0.5  i_specify=off  i_priority=None  i=0 A  i_nominal_specify=off  i_nominal_value=1  i_nominal_unit=A  v_specify=off  v_priority=None  v=0 V  v_nominal_specify=off  v_nominal_value=1  v_nominal_unit=V
  D : PMIOPort  Side=Left
  S : PMIOPort  Port=2  Side=Right
  wires:
  [gA_P5_S4] -> Gate_PS/1
  connections:
  Gate_PS/RConn1 -- SW/RConn1
  SW/LConn1 -- D/RConn1 -- D_body/RConn1 -- C_oss/LConn1
  SW/RConn2 -- D_body/LConn1 -- S/RConn1 -- C_oss/RConn1

== system TB32_A25R_ClampMix/StageA_Module3/StageA_Phase6/S1_VIN_A ==
  note: 스위치 셀: 이상 스위치(R_on, G_off) + 역병렬 바디 다이오드(Vf, R_d) + 출력용량 C_oss
      | 게이트: 전역 태그 "gA_P6_S1" (> 0.5 이면 도통)
  C_oss : fl_lib/Electrical/Electrical Elements/Capacitor  c=Coss F  r=1e-6 Ohm  g=0 1/Ohm  i_specify=off  i_priority=None  i=0 A  i_nominal_specify=off  i_nominal_value=1  i_nominal_unit=A  v_specify=off  v_priority=None  v=0 V  v_nominal_specify=off  v_nominal_value=1  v_nominal_unit=V  vc_specify=off  vc_priority=High  vc=0 V  vc_nominal_specify=off  vc_nominal_value=1  vc_nominal_unit=V
  D_body : fl_lib/Electrical/Electrical Elements/Diode  Vf=Vf V  Ron=Rd Ohm  Goff=Goffd 1/Ohm  i_specify=off  i_priority=None  i=0 A  i_nominal_specify=off  i_nominal_value=1  i_nominal_unit=A  v_specify=off  v_priority=None  v=0 V  v_nominal_specify=off  v_nominal_value=1  v_nominal_unit=V
  Gate_PS : nesl_utility/Simulink-PS Converter  PhysicalDomain=network_engine_domain  SubClassName=ps_input  LeftPortType=input  RightPortType=output  PseudoPeriodic=off  Frequencies=[]  NoiseDistribution=none  NoiseParameters=[]  Unit=1  AffineConversion=off  FilteringAndDerivatives=zero  SimscapeFilterOrder=1  InputFilterTimeConstant=0.001  UdotUserProvided=0
  SW : fl_lib/Electrical/Electrical Elements/Switch  R_closed=Ron Ohm  G_open=Goff 1/Ohm  Threshold=0.5  i_specify=off  i_priority=None  i=0 A  i_nominal_specify=off  i_nominal_value=1  i_nominal_unit=A  v_specify=off  v_priority=None  v=0 V  v_nominal_specify=off  v_nominal_value=1  v_nominal_unit=V
  D : PMIOPort  Side=Left
  S : PMIOPort  Port=2  Side=Right
  wires:
  [gA_P6_S1] -> Gate_PS/1
  connections:
  Gate_PS/RConn1 -- SW/RConn1
  SW/LConn1 -- D/RConn1 -- D_body/RConn1 -- C_oss/LConn1
  SW/RConn2 -- D_body/LConn1 -- S/RConn1 -- C_oss/RConn1
